simulink library "pgtrafo"  (R2016b)
settings: Solver=VariableStepAuto  StartTime=0.0  StopTime=10.0  RelTol=1e-3
undefined symbols (not defined in the file or in its folder): R3, SO3
libraries: pgtrafo x9, pgmanif x3, pgctrl x1, simulink_need_slupdate x1
settings Model: Creator=mueh_mm  LastModifiedBy=mueh_mm

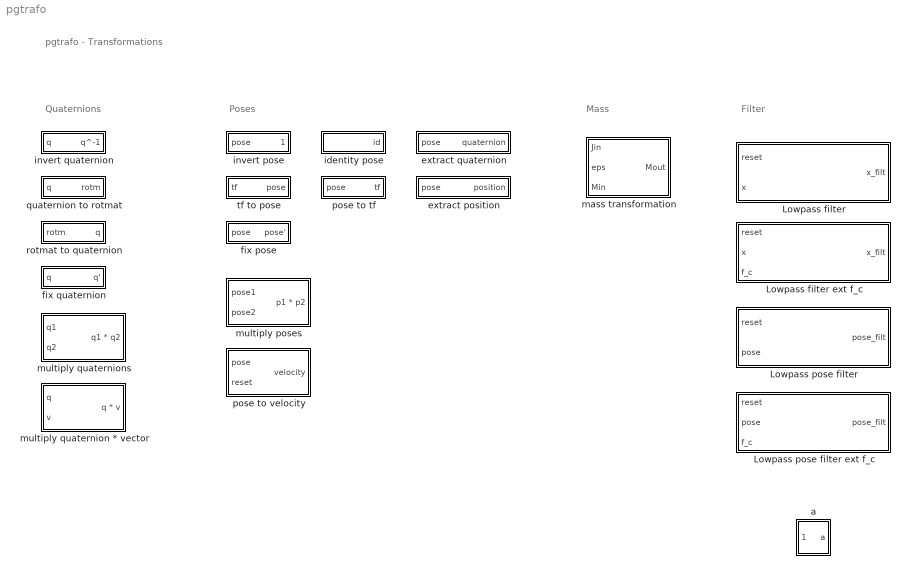
== system pgtrafo ==
  note: pgtrafo - Transformations
  note: Quaternions
  note: Poses
  note: Mass
  note: Filter
  Lowpass filter : Subsystem  mask(Lowpass Filter){f_c=30}
      mask prompts: f_c "Cutoff Frequency"
      mask help: This block implements a lowpass filter with cutoff frequency f_c.
      mask Display:
      | disp(['Cutoff: ' num2str(f_c) 'Hz']);
      | port_label('input', 1, 'reset');
      | port_label('input', 2, 'x');
      | port_label('output', 1, 'x_filt');
  Lowpass filter ext f_c : Subsystem  mask(Lowpass Filter){}
      mask help: This block implements a lowpass filter with cutoff frequency f_c.
      mask Display:
      | disp(['Lowpass']);
      | port_label('input', 1, 'reset');
      | port_label('input', 2, 'x');
      | port_label('input', 3, 'f_c');
      | port_label('output', 1, 'x_filt');
  Lowpass pose filter : Subsystem  mask(Lowpass filter){f_c=30}
      mask prompts: f_c "Cutoff Frequency"
      mask help: This block implements lowpass filtering of a pose.
      mask Display:
      | disp(['Cutoff: ' num2str(f_c) 'Hz']);
      | port_label('input', 1, 'reset');
      | port_label('input', 2, 'pose');
      | port_label('output', 1, 'pose_filt');
  Lowpass pose filter ext f_c : Subsystem  mask(Lowpass filter){f_c=30}
      mask prompts: f_c "Cutoff Frequency"
      mask help: This block implements lowpass filtering of a pose.
      mask Display:
      | disp(['Cutoff: ' num2str(f_c) 'Hz']);
      | port_label('input', 1, 'reset');
      | port_label('input', 2, 'pose');
      | port_label('input', 3, 'f_c');
      | port_label('output', 1, 'pose_filt');
  a : Subsystem
  extract position : Subsystem
  extract quaternion : Subsystem
  fix pose : Subsystem
  fix quaternion : Subsystem
  identity pose : Subsystem
  invert pose : Subsystem
  invert quaternion : Subsystem
  mass transformation : Subsystem
  multiply poses : Subsystem
  multiply quaternion * vector : Subsystem
  multiply quaternions : Subsystem
  pose to tf : Subsystem
  pose to velocity : Subsystem
  quaternion to rotmat : Subsystem
  rotmat to quaternion : Subsystem
  tf to pose : Subsystem

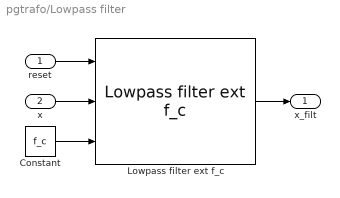
== system pgtrafo/Lowpass filter ==
  reset : Inport
  x : Inport  Port=2
  Constant : Constant  Value=f_c
  Lowpass filter ext f_c : pgtrafo/Lowpass filter ext f_c
  x_filt : Outport
  wires:
  Lowpass filter ext f_c/1 -> x_filt/1
  x/1 -> Lowpass filter ext f_c/2
  reset/1 -> Lowpass filter ext f_c/1
  Constant/1 -> Lowpass filter ext f_c/3

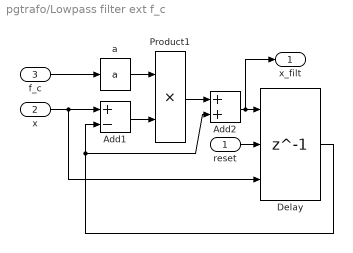
== system pgtrafo/Lowpass filter ext f_c ==
  reset : Inport
  x : Inport  Port=2
  f_c : Inport  Port=3
  Add1 : Sum  Inputs=+-
  Add2 : Sum
  Delay : Delay  DelayLength=1  InitialConditionSource=Input port  ExternalReset=Either
      settings: InputPortMap=u0,r5,p4
  Product1 : Product
  a : pgtrafo/a
  x_filt : Outport
  wires:
  x/1 -> Delay/3, Add1/1
  Delay/1 -> Add2/2, Add1/2
  reset/1 -> Delay/2
  Add1/1 -> Product1/2
  Product1/1 -> Add2/1
  Add2/1 -> Delay/1, x_filt/1
  a/1 -> Product1/1
  f_c/1 -> a/1

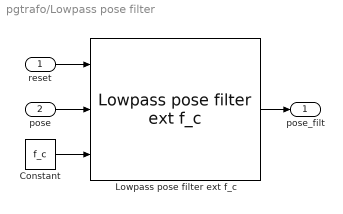
== system pgtrafo/Lowpass pose filter ==
  reset : Inport
  pose : Inport  Port=2
  Constant : Constant  Value=f_c
  Lowpass pose filter ext f_c : pgtrafo/Lowpass pose filter ext f_c  f_c=30
  pose_filt : Outport
  wires:
  pose/1 -> Lowpass pose filter ext f_c/2
  reset/1 -> Lowpass pose filter ext f_c/1
  Constant/1 -> Lowpass pose filter ext f_c/3
  Lowpass pose filter ext f_c/1 -> pose_filt/1

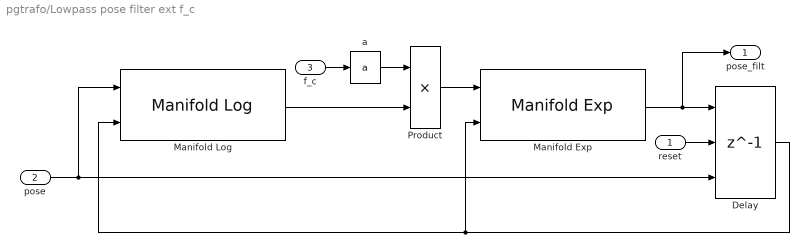
== system pgtrafo/Lowpass pose filter ext f_c ==
  reset : Inport
  pose : Inport  Port=2
  f_c : Inport  Port=3
  Delay : Delay  DelayLength=1  InitialConditionSource=Input port  ExternalReset=Either
      settings: InputPortMap=u0,r5,p4
  Manifold Exp : pgmanif/Manifold Exp  manifold_description_raw=R3*SO3  manifold_description=0  dim_manifold=0  dim_tangent=0
  Manifold Log : pgmanif/Manifold Log  manifold_description_raw=R3*SO3  manifold_description=0  dim_manifold=0  dim_tangent=0
  Product : Product
  a : pgtrafo/a
  pose_filt : Outport
  wires:
  Manifold Log/1 -> Product/2
  a/1 -> Product/1
  Product/1 -> Manifold Exp/1
  Delay/1 -> Manifold Exp/2, Manifold Log/2
  pose/1 -> Delay/3, Manifold Log/1
  Manifold Exp/1 -> Delay/1, pose_filt/1
  reset/1 -> Delay/2
  f_c/1 -> a/1

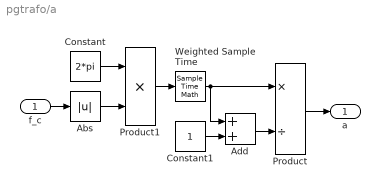
== system pgtrafo/a ==
  f_c : Inport
  Abs : Abs
  Add : Sum
  Constant : Constant  Value=2*pi
  Constant1 : Constant
  Product : Product  Inputs=*/
  Product1 : Product
  Weighted Sample Time : SampleTimeMath  TsampMathOp=*
  a : Outport
  wires:
  Constant1/1 -> Add/2
  Product/1 -> a/1
  Constant/1 -> Product1/1
  Add/1 -> Product/2
  Weighted Sample Time/1 -> Product/1, Add/1
  Product1/1 -> Weighted Sample Time/1
  Abs/1 -> Product1/2
  f_c/1 -> Abs/1

== system pgtrafo/extract position ==
  pose : Inport
  Position : Selector  InputPortWidth=7  IndexOptions=Index vector (dialog)  Indices=1:3  OutputSizes=1
  position : Outport
  wires:
  pose/1 -> Position/1
  Position/1 -> position/1

== system pgtrafo/extract quaternion ==
  pose : Inport
  Quaternion : Selector  InputPortWidth=7  IndexOptions=Index vector (dialog)  Indices=4:7  OutputSizes=1
  quaternion : Outport
  wires:
  Quaternion/1 -> quaternion/1
  pose/1 -> Quaternion/1

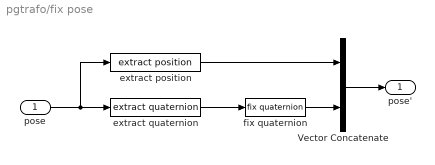
== system pgtrafo/fix pose ==
  pose : Inport
  Vector Concatenate : Concatenate
  extract position : pgtrafo/extract position
  extract quaternion : pgtrafo/extract quaternion
  fix quaternion : pgtrafo/fix quaternion
  pose' : Outport
  wires:
  pose/1 -> extract quaternion/1, extract position/1
  extract quaternion/1 -> fix quaternion/1
  fix quaternion/1 -> Vector Concatenate/2
  extract position/1 -> Vector Concatenate/1
  Vector Concatenate/1 -> pose'/1

== system pgtrafo/fix quaternion ==
  q : Inport
  quaternion fix : MATLAB Function  TreatAsAtomicUnit=on
  q' : Outport
  wires:
  q/1 -> quaternion fix/1(q)
  quaternion fix/1(qfix) -> q'/1

== system pgtrafo/identity pose ==
  Constant : Constant  Value=[0 0 0 0 0 0 1]
  id : Outport
  wires:
  Constant/1 -> id/1

== system pgtrafo/invert pose ==
  pose : Inport
  Pose Inversion : MATLAB Function  TreatAsAtomicUnit=on
  pose^-1 : Outport
  wires:
  pose/1 -> Pose Inversion/1(p)
  Pose Inversion/1(res) -> pose^-1/1

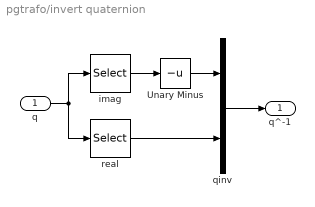
== system pgtrafo/invert quaternion ==
  q : Inport
  Unary Minus : UnaryMinus
  imag : Selector  InputPortWidth=4  IndexOptions=Index vector (dialog)  Indices=1:3  OutputSizes=1
  qinv : Concatenate
  real : Selector  InputPortWidth=4  IndexOptions=Index vector (dialog)  Indices=4  OutputSizes=1
  q^-1 : Outport
  wires:
  real/1 -> qinv/2
  Unary Minus/1 -> qinv/1
  imag/1 -> Unary Minus/1
  q/1 -> imag/1, real/1
  qinv/1 -> q^-1/1

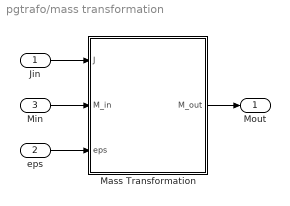
== system pgtrafo/mass transformation ==
  Jin : Inport
  eps : Inport  Port=2
  Min : Inport  Port=3
  Mass Transformation : MATLAB Function  TreatAsAtomicUnit=on
  Mout : Outport
  wires:
  Min/1 -> Mass Transformation/2(M_in)
  Jin/1 -> Mass Transformation/1(J)
  Mass Transformation/1(M_out) -> Mout/1
  eps/1 -> Mass Transformation/3(eps)

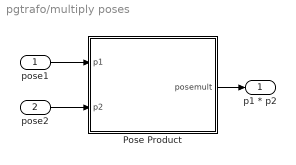
== system pgtrafo/multiply poses ==
  pose1 : Inport
  pose2 : Inport  Port=2
  Pose Product : MATLAB Function  TreatAsAtomicUnit=on
  p1 * p2 : Outport
  wires:
  Pose Product/1(posemult) -> p1 * p2/1
  pose1/1 -> Pose Product/1(p1)
  pose2/1 -> Pose Product/2(p2)

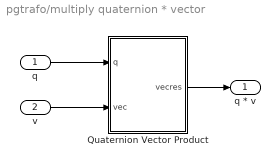
== system pgtrafo/multiply quaternion * vector ==
  q : Inport
  v : Inport  Port=2
  Quaternion Vector Product : MATLAB Function  TreatAsAtomicUnit=on
  q * v : Outport
  wires:
  Quaternion Vector Product/1(vecres) -> q * v/1
  q/1 -> Quaternion Vector Product/1(q)
  v/1 -> Quaternion Vector Product/2(vec)

== system pgtrafo/multiply quaternions ==
  q1 : Inport
  q2 : Inport  Port=2
  Quaternion Product : MATLAB Function  TreatAsAtomicUnit=on
  q1 * q2 : Outport
  wires:
  q1/1 -> Quaternion Product/1(q1)
  q2/1 -> Quaternion Product/2(q2)
  Quaternion Product/1(qmult) -> q1 * q2/1

== system pgtrafo/pose to tf ==
  pose : Inport
  Pose To Tf : MATLAB Function  TreatAsAtomicUnit=on
  Selector : Selector  NumberOfDimensions=2  InputPortWidth=3  IndexOptions=Index vector (dialog),Select all  Indices=1:3,1  OutputSizes=1,1
  tf : Outport
  wires:
  pose/1 -> Pose To Tf/1(p)
  Pose To Tf/1(tf) -> Selector/1
  Selector/1 -> tf/1

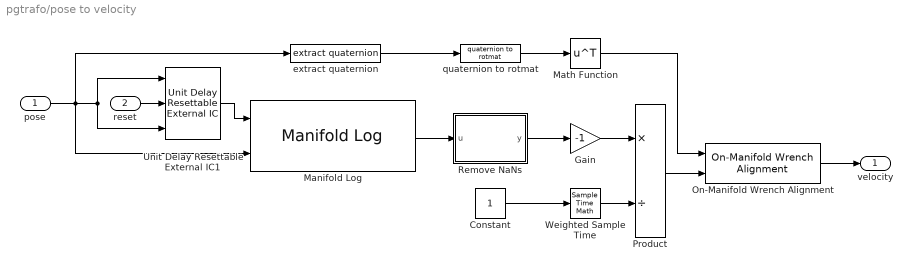
== system pgtrafo/pose to velocity ==
  pose : Inport
  reset : Inport  Port=2
  Constant : Constant
  Gain : Gain  Gain=-1
  Manifold Log : pgmanif/Manifold Log  manifold_description_raw=R3*SO3  manifold_description=0  dim_manifold=0  dim_tangent=0
  Math Function : Math  Operator=transpose  SaturateOnIntegerOverflow=on
  On-Manifold Wrench Alignment : pgctrl/On-Manifold Wrench Alignment
  Product : Product  Inputs=*/
  Remove NaNs : MATLAB Function  TreatAsAtomicUnit=on
  Unit Delay Resettable External IC1 : simulink_need_slupdate/Unit Delay Resettable External IC  tsamp=-1
  Weighted Sample Time : SampleTimeMath  TsampMathOp=*  weightValue=1  TsampMathImp=Offline Scaling Adjustment
  extract quaternion : pgtrafo/extract quaternion
  quaternion to rotmat : pgtrafo/quaternion to rotmat
  velocity : Outport
  wires:
  pose/1 -> Unit Delay Resettable External IC1/1, Unit Delay Resettable External IC1/3, extract quaternion/1, Manifold Log/2
  Manifold Log/1 -> Remove NaNs/1(u)
  Remove NaNs/1(y) -> Gain/1
  Gain/1 -> Product/1
  Unit Delay Resettable External IC1/1 -> Manifold Log/1
  Constant/1 -> Weighted Sample Time/1
  Weighted Sample Time/1 -> Product/2
  On-Manifold Wrench Alignment/1 -> velocity/1
  Product/1 -> On-Manifold Wrench Alignment/2
  quaternion to rotmat/1 -> Math Function/1
  extract quaternion/1 -> quaternion to rotmat/1
  Math Function/1 -> On-Manifold Wrench Alignment/1
  reset/1 -> Unit Delay Resettable External IC1/2

== system pgtrafo/quaternion to rotmat ==
  q : Inport
  q to rotm : MATLAB Function  TreatAsAtomicUnit=on
  rotm : Outport
  wires:
  q/1 -> q to rotm/1(q)
  q to rotm/1(rotm) -> rotm/1

== system pgtrafo/rotmat to quaternion ==
  rotm : Inport
  rotm to q : MATLAB Function  TreatAsAtomicUnit=on
  q : Outport
  wires:
  rotm to q/1(q) -> q/1
  rotm/1 -> rotm to q/1(rotm)

== system pgtrafo/tf to pose ==
  tf : Inport
  Tf 2 Pose : MATLAB Function  TreatAsAtomicUnit=on
  pose : Outport
  wires:
  Tf 2 Pose/1(p) -> pose/1
  tf/1 -> Tf 2 Pose/1(tf)

== matlab function pgtrafo/mass transformation/Mass Transformation ==
  data: J input; M_out output; M_in input; eps input
function M_out = mass_transformation(J, M_in, eps)
% J transforms velocities in in to velocities in out

M_out = (J * M_in^-1 * J' + eps*eye(6))^-1;

== matlab function pgtrafo/rotmat to quaternion/rotm to q ==
  data: rotm input; q output
function q = rotm2quat(rotm)

q = pglfd.geom.so3.rotmat_to_quaternion(rotm);

== matlab function pgtrafo/multiply quaternions/Quaternion Product ==
  data: q1 input; qmult output; q2 input
function qmult = qprod(q1, q2)

qmult = pglfd.geom.so3.quaternion_multiply(q1, q2);

== matlab function pgtrafo/pose to velocity/Remove NaNs ==
  data: u input; y output
function y = remove_nans(u)

y = u;

% replace all non finite values by 0's
y(~isfinite(y)) = 0;

== matlab function pgtrafo/quaternion to rotmat/q to rotm ==
  data: q input; rotm output
function rotm = quat2rotm(q)

rotm = pglfd.geom.so3.quaternion_to_rotmat(q);

== matlab function pgtrafo/fix quaternion/quaternion fix ==
  data: q input; qfix output
function qfix = quatfix(q)

qfix = pglfd.geom.so3.quaternion_fix(q);

== matlab function pgtrafo/multiply quaternion * vector/Quaternion Vector Product ==
  data: q input; vecres output; vec input
function vecres = vecprod(q, vec)

vecres = pglfd.geom.so3.quaternion_vector_multiply(q, vec);

== matlab function pgtrafo/invert pose/Pose Inversion ==
  data: p input; res output
function res = pose_inversion(p)

res = pglfd.geom.se3.pose_inversion(p);

== matlab function pgtrafo/multiply poses/Pose Product ==
  data: p1 input; posemult output; p2 input
function posemult = poseprod(p1, p2)

posemult = pglfd.geom.se3.pose_multiply(p1, p2);

== matlab function pgtrafo/pose to tf/Pose To Tf ==
  data: p input; tf output
function tf = pose_to_tf(p)

tf = pglfd.geom.se3.pose_to_tf(p);

== matlab function pgtrafo/tf to pose/Tf 2 Pose ==
  data: tf input; p output
function p = tf_to_pose(tf)

p = pglfd.geom.se3.tf_to_pose(tf);
